simulink model "Pressure_actuationOnly"  (R2025a)
settings: Solver=FixedStepAuto  StartTime=0.0  StopTime=inf  FixedStep=1/100  RelTol=1e-3
model workspace (MAT data in the model file):
  W1_l1 = [-0.00637147299334 -0.00624802223118 -0.00619603187657 0.00818749930186 -0.00424511993807 -0.00083745726232 -0.00833424331717 0.00697799997251 -0.00715003670843 -0.00626604831718 -0.0705428701228 0.00662881038519 ... (5376 elements, 64x84)]
  W1_l2 = [0 0 0 0 0 0 0 0 0 0 0 0 ... (5376 elements, 64x84)]
  W1_l3 = [0 0 0 0 0 0 0 0 0 0 0 0 ... (5376 elements, 64x84)]
  W2_l1 = [-0.0156497886645 0.016762621794 0.0167348569836 -0.0231262161799 0.0185108770145 -0.0187268245245 -0.014776023883 0.0177292072634 -0.013613498126 0.0173024291583 0.0215678825224 0.0115265826162 ... (2048 elements, 32x64)]
  W2_l2 = [-0.0377476122839 0.0538729387073 0.0438303187069 0.0464086258401 -0.0417546570682 0.011838804868 -0.0417271960925 0.0426008315381 -0.0444773085117 0.0424451718893 -0.040141386682 -0.0533310100989 ... (2048 elements, 32x64)]
  W2_l3 = [-0.00361323771562 0.0123768179777 0.0107080464844 0.0199177209848 -0.0177829565655 0.00824623343895 -0.00619824742788 -0.00214531281672 0.0148743772087 0.01947258566 0.00407370811971 -0.0163192085678 ... (2048 elements, 32x64)]
  W3_l1 = [0.132052254619 -0.375379893145 -0.446932223908 0.357797717849 -0.393217065478 0.411103098765 0.371578024157 -0.337760153494 0.140027914221 -0.315977756494 -0.307174196243 -0.120115030619 ... (32 elements, 1x32)]
  W3_l2 = [0.279554184021 -0.471512064684 -0.325051298271 -0.35734053232 0.304912543396 -0.0794739072662 0.308632495485 -0.320908393214 0.332378526357 -0.310167970162 0.29099894839 0.446829975634 ... (32 elements, 1x32)]
  W3_l3 = [-0.0570001238091 0.199424322924 0.209089111533 0.603627643255 -0.418786165651 0.0997717774498 -0.0840156243336 -0.0236237427471 0.379327938099 0.50292362288 0.0108831688655 -0.34227191869 ... (32 elements, 1x32)]
  b1_l1 = [0.00710175645196 0.000369184720508 0.000710181990281 0.0393455266092 0.00950708970836 0.0109777156356 -0.0133124765123 -0.00522158774426 0.00164422558321 0.00576255868365 -0.0478743336823 -0.00160511772982 ... (64 elements, 64x1)]
  b1_l2 = [-0.0147426613482 -0.00869580439207 0.0138765328616 0.0138284489813 0.000295621534183 0.00725342474904 -0.0162273626443 0.0446493349263 -0.0905339713803 -0.00601908350527 0.00965038861913 0.0030522537524 ... (64 elements, 64x1)]
  b1_l3 = [-0.000999045790686 0.000698575449992 -0.000605690473725 0.00160280732153 0.000523282728528 -0.00213430900699 0.0122687697595 0.0390874045108 -0.00278736371045 9.98305151793e-05 -0.0103509580715 -0.00835315937259 ... (64 elements, 64x1)]
  b2_l1 = [-0.000401046663753 -0.00628788563213 -0.0346303888099 -0.00586372666504 -0.00699317952995 0.0114299600793 0.00801395570366 9.06123695651e-06 -0.00162311128817 0.00111045782214 0.00577555943279 0.00114995118652 ... (32 elements, 32x1)]
  b2_l2 = [-0.00687229898615 -0.0142918895776 7.1088213054e-05 0.000748920257724 -0.00405581737759 0.00582158552269 -0.00525058718115 0.000648576074579 -0.00268108657353 0.00285048552601 -0.00419904310146 0.00427594767426 ... (32 elements, 32x1)]
  b2_l3 = [0.000387927607183 -0.00245267007242 0.00370637057149 0.0310088937782 -0.0366301531366 -0.00271870043869 0.00169361465885 0.000929703220207 0.0102090594854 0.0356739380334 -0.00594828418232 0.000255561344574 ... (32 elements, 32x1)]
  b3_l1 = -0.00698359211629
  b3_l2 = -0.0434220447048
  b3_l3 = 0.00285349149877
  muX_l1 = [1.57694541084 0 0 -0.00336127639137 0 0 0.0206891205991 0 0 1.57697902361 0 0 ... (84 elements, 84x1)]
  muX_l2 = [0 1.57694541084 0 0 -0.00336127639137 0 0 0.0206891205991 0 0 1.57697902361 0 ... (84 elements, 84x1)]
  muX_l3 = [0 0 1.57694541084 0 0 -0.00336127639137 0 0 0.0206891205991 0 0 1.57697902361 ... (84 elements, 84x1)]
  muY_l1 = 0.0157844107063
  muY_l2 = 0.0112303577139
  muY_l3 = 0.0148868176685
  sigX_l1 = [1.05565395992 1e-08 1e-08 4.060486428 1e-08 1e-08 0.995838667948 1e-08 1e-08 1.0556525752 1e-08 1e-08 ... (84 elements, 84x1)]
  sigX_l2 = [1e-08 1.05565395992 1e-08 1e-08 4.060486428 1e-08 1e-08 0.995838667948 1e-08 1e-08 1.0556525752 1e-08 ... (84 elements, 84x1)]
  sigX_l3 = [1e-08 1e-08 1.05565395992 1e-08 1e-08 4.060486428 1e-08 1e-08 0.995838667948 1e-08 1e-08 1.0556525752 ... (84 elements, 84x1)]
  sigY_l1 = 0.0111510578581
  sigY_l2 = 0.00895432840902
  sigY_l3 = 0.0121006138289
undefined symbols (not defined in the file or in its folder): National_Instruments, PCI
libraries: sldrtlib x3
(part 2 of 2)

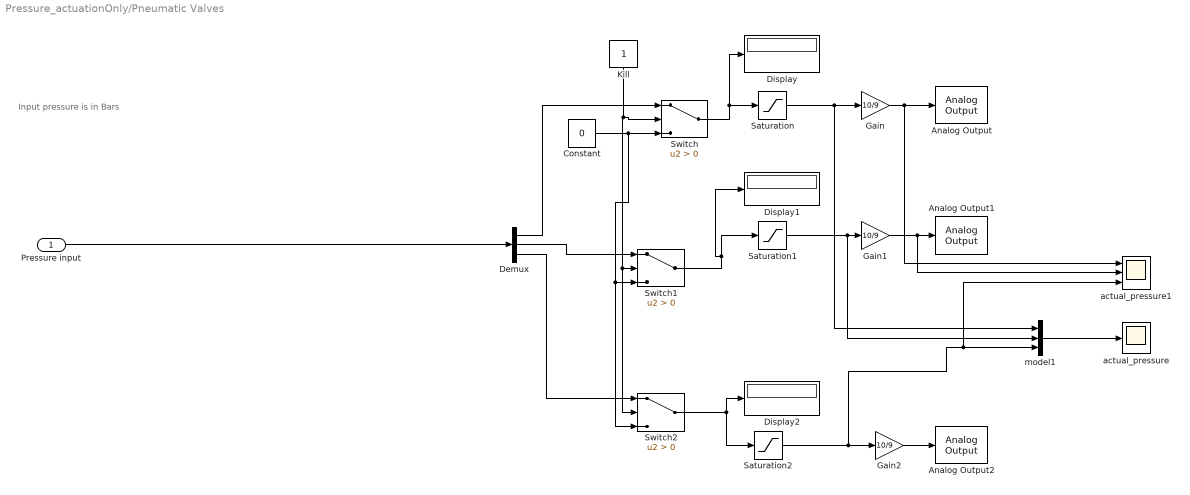
== system Pressure_actuationOnly/Pneumatic Valves ==
  note: Input pressure is in Bars
  Pressure input : Inport
  Analog Output : sldrtlib/Analog Output  SampleTime=1/100  MaxMissedTicks=inf  ShowMissedTicks=off  YieldWhenWaiting=on  DrvName=National_Instruments/PCI-6703  DrvAddress=4294967295  DrvOptions=0  Channels=1  RangeMode=1  VoltRange=1  InitialValue=0  FinalValue=0
      settings: AttributesFormatString=National Instruments\nPCI-6703 [auto]
  Analog Output1 : sldrtlib/Analog Output  SampleTime=1/100  MaxMissedTicks=inf  ShowMissedTicks=off  YieldWhenWaiting=off  DrvName=National_Instruments/PCI-6703  DrvAddress=4294967295  DrvOptions=0  Channels=2  RangeMode=1  VoltRange=1  InitialValue=0  FinalValue=0
      settings: AttributesFormatString=National Instruments\nPCI-6703 [auto]
  Analog Output2 : sldrtlib/Analog Output  SampleTime=1/100  MaxMissedTicks=inf  ShowMissedTicks=off  YieldWhenWaiting=off  DrvName=National_Instruments/PCI-6703  DrvAddress=4294967295  DrvOptions=0  Channels=3  RangeMode=1  VoltRange=1  InitialValue=0  FinalValue=0
      settings: AttributesFormatString=National Instruments\nPCI-6703 [auto]
  Constant : Constant  Value=0
  Demux : Demux  Outputs=3
  Display : Display
  Display1 : Display
  Display2 : Display
  Gain : Gain  Gain=10/9
  Gain1 : Gain  Gain=10/9
  Gain2 : Gain  Gain=10/9
  Kill : Constant
  Saturation : Saturate  UpperLimit=3  LowerLimit=0
  Saturation1 : Saturate  UpperLimit=3  LowerLimit=0
  Saturation2 : Saturate  UpperLimit=3  LowerLimit=0
  Switch : Switch  Criteria=u2 > Threshold  SaturateOnIntegerOverflow=off  InputSameDT=off
  Switch1 : Switch  Criteria=u2 > Threshold  SaturateOnIntegerOverflow=off  InputSameDT=off
  Switch2 : Switch  Criteria=u2 > Threshold  SaturateOnIntegerOverflow=off  InputSameDT=off
  actual_pressure : Scope
      settings: ActiveDisplayYMinimum=-0.37499999999999989  ActiveDisplayYMaximum=3.375  DataLoggingVariableName=ScopeData7
  actual_pressure1 : Scope  NumInputPorts=3
      settings: ActiveDisplayYMinimum=-0.37499999999999989  ActiveDisplayYMaximum=3.375
  model1 : Mux  Inputs=3
  wires:
  Constant/1 -> Switch2/3, Switch1/3, Switch/3
  Kill/1 -> Switch2/2, Switch1/2, Switch/2
  Switch/1 -> Display/1, Saturation/1
  Gain/1 -> actual_pressure1/1, Analog Output/1
  Saturation/1 -> model1/1, Gain/1
  Demux/3 -> Switch2/1
  Gain1/1 -> actual_pressure1/2, Analog Output1/1
  Gain2/1 -> Analog Output2/1
  Saturation2/1 -> actual_pressure1/3, model1/3, Gain2/1
  Switch2/1 -> Saturation2/1, Display2/1
  Demux/2 -> Switch1/1
  Switch1/1 -> Saturation1/1, Display1/1
  model1/1 -> actual_pressure/1
  Saturation1/1 -> model1/2, Gain1/1
  Demux/1 -> Switch/1
  Pressure input/1 -> Demux/1
